simulink model "baseline_ideal_switching_open_loop"  (R2023b)
settings: Solver=ode4  StartTime=0.0  StopTime=0.23999999999999999  FixedStep=4.9999999999999998e-07  RelTol=1e-3
Description:
  | Stage 0 baseline: ideal unipolar SPWM switching function plus continuous LC state equations. Open loop. No dead time or device loss.
settings Model: Creator=Oll1ver  LastModifiedBy=Oll1ver
settings DataIOCC: SaveOutput=off  SaveTime=off

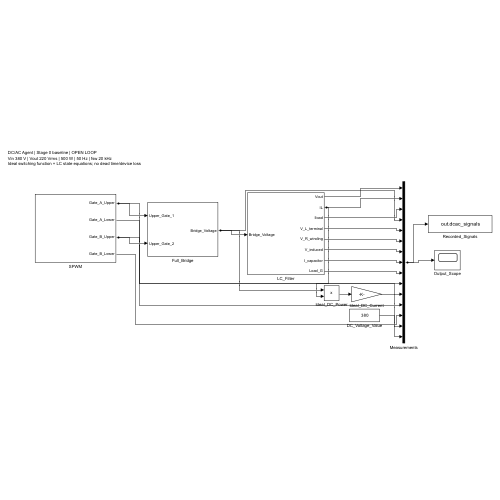
[thumbnail: Simulink's stored preview of the top-level diagram]
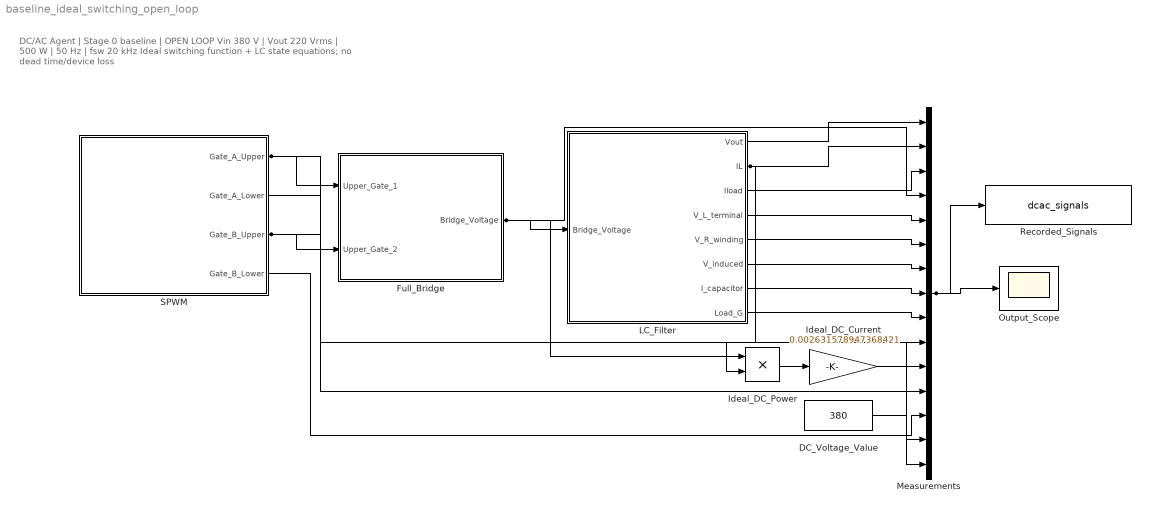
== system baseline_ideal_switching_open_loop ==
  note: DC/AC Agent | Stage 0 baseline | OPEN LOOP
      | Vin 380 V | Vout 220 Vrms | 500 W | 50 Hz | fsw 20 kHz
      | Ideal switching function + LC state equations; no dead time/device loss
  DC_Voltage_Value : Constant  Value=380
  Full_Bridge : Subsystem
  Ideal_DC_Current : Gain  Gain=0.002631578947368421
  Ideal_DC_Power : Product
  LC_Filter : Subsystem
  Measurements : Mux  Inputs=15
  Output_Scope : Scope
  Recorded_Signals : ToWorkspace  VariableName=dcac_signals  SaveFormat=Timeseries  SampleTime=-1
  SPWM : Subsystem
  wires:
  SPWM/1(Gate_A_Upper) -> Full_Bridge/1(Upper_Gate_1), Measurements/10
  SPWM/3(Gate_B_Upper) -> Full_Bridge/2(Upper_Gate_2), Measurements/12
  Full_Bridge/1(Bridge_Voltage) -> LC_Filter/1(Bridge_Voltage), Ideal_DC_Power/1, Measurements/4
  LC_Filter/2(IL) -> Ideal_DC_Power/2, Measurements/2
  Ideal_DC_Power/1 -> Ideal_DC_Current/1
  LC_Filter/1(Vout) -> Measurements/1
  LC_Filter/3(Iload) -> Measurements/3
  LC_Filter/4(V_L_terminal) -> Measurements/5
  LC_Filter/5(V_R_winding) -> Measurements/6
  LC_Filter/6(V_induced) -> Measurements/7
  LC_Filter/7(I_capacitor) -> Measurements/8
  LC_Filter/8(Load_G) -> Measurements/9
  SPWM/2(Gate_A_Lower) -> Measurements/11
  SPWM/4(Gate_B_Lower) -> Measurements/13
  Ideal_DC_Current/1 -> Measurements/14
  DC_Voltage_Value/1 -> Measurements/15
  Measurements/1 -> Recorded_Signals/1, Output_Scope/1

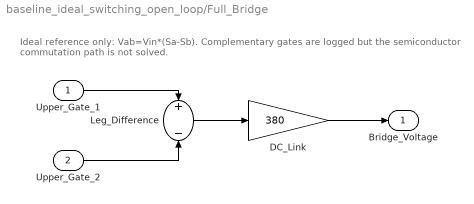
== system baseline_ideal_switching_open_loop/Full_Bridge ==
  note: Ideal reference only: Vab=Vin*(Sa-Sb). Complementary gates are logged but the semiconductor commutation path is not solved.
  Upper_Gate_1 : Inport
  Upper_Gate_2 : Inport  Port=2
  DC_Link : Gain  Gain=380
  Leg_Difference : Sum  Inputs=+-
  Bridge_Voltage : Outport
  wires:
  Upper_Gate_1/1 -> Leg_Difference/1
  Upper_Gate_2/1 -> Leg_Difference/2
  Leg_Difference/1 -> DC_Link/1
  DC_Link/1 -> Bridge_Voltage/1

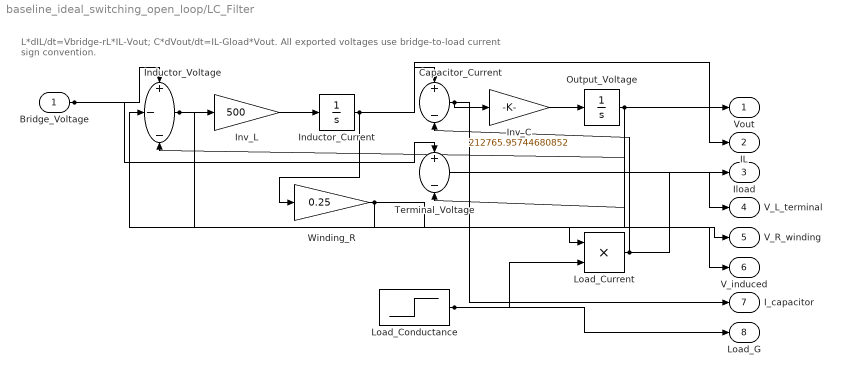
== system baseline_ideal_switching_open_loop/LC_Filter ==
  note: L*dIL/dt=Vbridge-rL*IL-Vout; C*dVout/dt=IL-Gload*Vout. All exported voltages use bridge-to-load current sign convention.
  Bridge_Voltage : Inport
  Capacitor_Current : Sum  Inputs=+-
  Inductor_Current : Integrator
  Inductor_Voltage : Sum  Inputs=+--
  Inv_C : Gain  Gain=212765.95744680852
  Inv_L : Gain  Gain=500
  Load_Conductance : Step  Time=0.12  Before=0.010330578512396695  After=0.010330578512396695  SampleTime=0
  Load_Current : Product
  Output_Voltage : Integrator
  Terminal_Voltage : Sum  Inputs=+-
  Winding_R : Gain  Gain=0.25
  Vout : Outport
  IL : Outport  Port=2
  Iload : Outport  Port=3
  V_L_terminal : Outport  Port=4
  V_R_winding : Outport  Port=5
  V_induced : Outport  Port=6
  I_capacitor : Outport  Port=7
  Load_G : Outport  Port=8
  wires:
  Bridge_Voltage/1 -> Inductor_Voltage/1, Terminal_Voltage/1
  Inductor_Voltage/1 -> Inv_L/1, V_induced/1
  Inv_L/1 -> Inductor_Current/1
  Inductor_Current/1 -> Winding_R/1, Capacitor_Current/1, IL/1
  Winding_R/1 -> Inductor_Voltage/2, V_R_winding/1
  Capacitor_Current/1 -> Inv_C/1, I_capacitor/1
  Inv_C/1 -> Output_Voltage/1
  Output_Voltage/1 -> Inductor_Voltage/3, Load_Current/1, Terminal_Voltage/2, Vout/1
  Load_Conductance/1 -> Load_Current/2, Load_G/1
  Load_Current/1 -> Capacitor_Current/2, Iload/1
  Terminal_Voltage/1 -> V_L_terminal/1

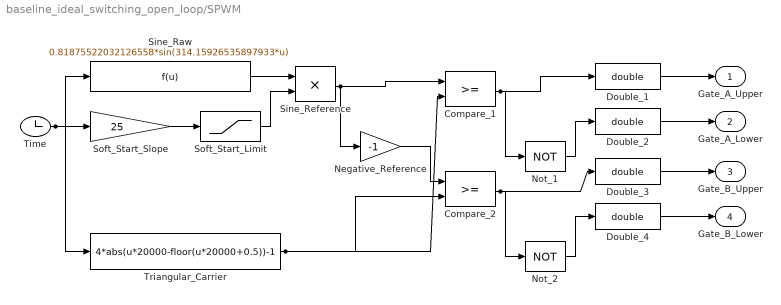
== system baseline_ideal_switching_open_loop/SPWM ==
  Compare_1 : RelationalOperator  OutDataTypeStr=boolean  RndMeth=Simplest  InputSameDT=off
  Compare_2 : RelationalOperator  OutDataTypeStr=boolean  RndMeth=Simplest  InputSameDT=off
  Double_{1..4} (4 alike) : DataTypeConversion  OutDataTypeStr=double  SaturateOnIntegerOverflow=off  RndMeth=Floor
  Negative_Reference : Gain  Gain=-1
  Not_1 : Logic  Operator=NOT  AllPortsSameDT=off  OutDataTypeStr=boolean
  Not_2 : Logic  Operator=NOT  AllPortsSameDT=off  OutDataTypeStr=boolean
  Sine_Raw : Fcn  Expr=0.81875522032126558*sin(314.15926535897933*u)
  Sine_Reference : Product
  Soft_Start_Limit : Saturate  UpperLimit=1  LowerLimit=0
  Soft_Start_Slope : Gain  Gain=25
  Time : Clock
  Triangular_Carrier : Fcn  Expr=4*abs(u*20000-floor(u*20000+0.5))-1
  Gate_A_Upper : Outport
  Gate_A_Lower : Outport  Port=2
  Gate_B_Upper : Outport  Port=3
  Gate_B_Lower : Outport  Port=4
  wires:
  Time/1 -> Triangular_Carrier/1, Sine_Raw/1, Soft_Start_Slope/1
  Soft_Start_Slope/1 -> Soft_Start_Limit/1
  Sine_Raw/1 -> Sine_Reference/1
  Soft_Start_Limit/1 -> Sine_Reference/2
  Sine_Reference/1 -> Negative_Reference/1, Compare_1/1
  Triangular_Carrier/1 -> Compare_1/2, Compare_2/2
  Compare_1/1 -> Not_1/1, Double_1/1
  Negative_Reference/1 -> Compare_2/1
  Compare_2/1 -> Not_2/1, Double_3/1
  Double_1/1 -> Gate_A_Upper/1
  Not_1/1 -> Double_2/1
  Double_2/1 -> Gate_A_Lower/1
  Double_3/1 -> Gate_B_Upper/1
  Not_2/1 -> Double_4/1
  Double_4/1 -> Gate_B_Lower/1
